simulink library "aerodynamics_lib"  (R2018b)
settings: Solver=VariableStepAuto  StartTime=0.0  StopTime=10.0  RelTol=1e-3
undefined symbols (not defined in the file): copterAero
settings Model: Creator=Ybeyer  LastModifiedBy=yannic
settings SFSimCC: SimUseLocalCustomCode=off
settings RTWCC: RTWUseLocalCustomCode=off
settings CodeAppCC: StateflowObjectComments=on

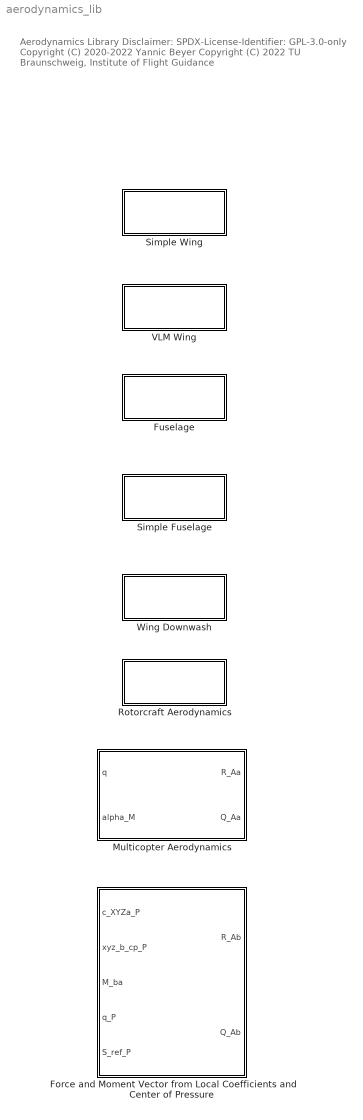
== system aerodynamics_lib ==
  note: Aerodynamics Library
      |
      | Disclaimer:
      | SPDX-License-Identifier: GPL-3.0-only
      |
      | Copyright (C) 2020-2022 Yannic Beyer
      | Copyright (C) 2022 TU Braunschweig, Institute of Flight Guidance
  Force and Moment Vector from Local Coefficients and Center of Pressure : MATLAB Function  TreatAsAtomicUnit=on
  Fuselage : Subsystem
      settings: OpenFcn=fuselage_lib
  Multicopter Aerodynamics : Subsystem  mask{S=copterAero.S, C_D_max=copterAero.C_Dmax, C_D_min=copterAero.C_Dmin, C_L_max=copterAero.C_Lmax, x_CoP_b=copterAero.CoP_xy, z_CoP_b=copterAero.CoP_z}
      mask prompts: S "reference area, m^2"; C_D_max "maximum drag coefficient, -"; C_D_min "minimum drag coefficient, -"; C_L_max "maximum lift coefficient, -"; x_CoP_b "x/y-distance of the center of pressure in body axes, m"; z_CoP_b "z position of the center of pressure in body axes, m"
      mask DialogControl DescGroupVar Prompt: Multicopter Aerodynamics
      mask DialogControl DescTextVar Prompt: This block computes the aerodynamic forces and moments of a simple quadcopter model. Please note that a modified definition of the aerodynamic angles is required.
      mask DialogControl Parameters Prompt: Parameters
  Rotorcraft Aerodynamics : Subsystem
      settings: OpenFcn=rotorcraft_lib
  Simple Fuselage : Subsystem
      settings: OpenFcn=simpleFuselage_lib
  Simple Wing : Subsystem
      settings: OpenFcn=simple_wing_lib
  VLM Wing : Subsystem
      settings: OpenFcn=vlm_wing_lib
  Wing Downwash : Subsystem
      settings: OpenFcn=wing_downwash_lib

== system aerodynamics_lib/Fuselage ==

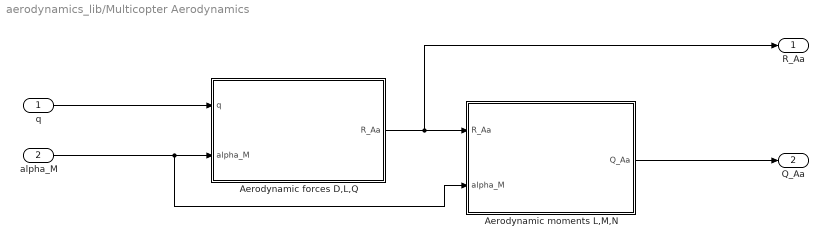
== system aerodynamics_lib/Multicopter Aerodynamics ==
  q : Inport
  alpha_M : Inport  Port=2
  Aerodynamic forces D,L,Q : Subsystem
  Aerodynamic moments L,M,N : Subsystem
  R_Aa : Outport
  Q_Aa : Outport  Port=2
  wires:
  q/1 -> Aerodynamic forces D,L,Q/1(q)
  alpha_M/1 -> Aerodynamic moments L,M,N/2(alpha_M), Aerodynamic forces D,L,Q/2(alpha_M)
  Aerodynamic moments L,M,N/1(Q_Aa) -> Q_Aa/1
  Aerodynamic forces D,L,Q/1(R_Aa) -> R_Aa/1, Aerodynamic moments L,M,N/1(R_Aa)

== system aerodynamics_lib/Rotorcraft Aerodynamics ==

== system aerodynamics_lib/Simple Fuselage ==

== system aerodynamics_lib/Simple Wing ==

== system aerodynamics_lib/VLM Wing ==

== system aerodynamics_lib/Wing Downwash ==

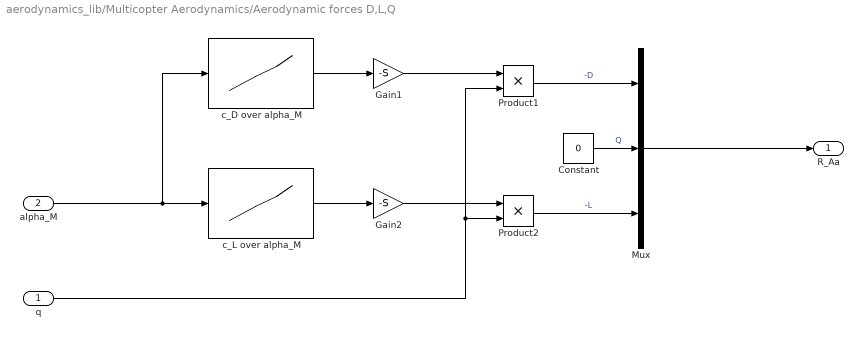
== system aerodynamics_lib/Multicopter Aerodynamics/Aerodynamic forces D,L,Q ==
  q : Inport
  alpha_M : Inport  Port=2
  Constant : Constant  Value=0
  Gain1 : Gain  Gain=-S
  Gain2 : Gain  Gain=-S
  Mux : Mux  Inputs=3
  Product1 : Product
  Product2 : Product
  c_D over alpha_M : Lookup_n-D  NumberOfTableDimensions=1  BreakpointsForDimension1=[-pi/2:pi/50:pi/2]  Table=(C_D_max-C_D_min)/2*-cos(-pi:pi/25:pi)+(C_D_max+C_D_min)/2  InternalRulePriority=Speed  RndMeth=Simplest  InputSameDT=on
  c_L over alpha_M : Lookup_n-D  NumberOfTableDimensions=1  BreakpointsForDimension1=[-pi/2:pi/50:pi/2]  Table=C_L_max*sin(-pi:pi/25:pi)  InternalRulePriority=Speed  RndMeth=Simplest  InputSameDT=on
  R_Aa : Outport
  wires:
  Gain1/1 -> Product1/1
  Mux/1 -> R_Aa/1
  Gain2/1 -> Product2/1
  Product2/1 -> Mux/3  "-L"
  c_D over alpha_M/1 -> Gain1/1
  c_L over alpha_M/1 -> Gain2/1
  alpha_M/1 -> c_D over alpha_M/1, c_L over alpha_M/1
  Product1/1 -> Mux/1  "-D"
  Constant/1 -> Mux/2  "Q"
  q/1 -> Product2/2, Product1/2

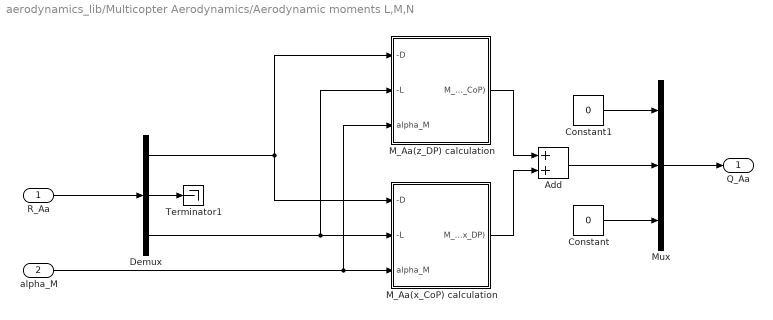
== system aerodynamics_lib/Multicopter Aerodynamics/Aerodynamic moments L,M,N ==
  R_Aa : Inport
  alpha_M : Inport  Port=2
  Add : Sum
  Constant : Constant  Value=0
  Constant1 : Constant  Value=0
  Demux : Demux  Outputs=3
  M_Aa(x_CoP) calculation : Subsystem
  M_Aa(z_DP) calculation : Subsystem
  Mux : Mux  Inputs=3
  Terminator1 : Terminator
  Q_Aa : Outport
  wires:
  Add/1 -> Mux/2
  M_Aa(x_CoP) calculation/1(M_Aa(x_DP)) -> Add/2
  M_Aa(z_DP) calculation/1(M_Aa(z_CoP)) -> Add/1
  Demux/3 -> M_Aa(z_DP) calculation/2(-L), M_Aa(x_CoP) calculation/2(-L)
  alpha_M/1 -> M_Aa(z_DP) calculation/3(alpha_M), M_Aa(x_CoP) calculation/3(alpha_M)
  Demux/1 -> M_Aa(z_DP) calculation/1(-D), M_Aa(x_CoP) calculation/1(-D)
  Demux/2 -> Terminator1/1
  Constant/1 -> Mux/3
  R_Aa/1 -> Demux/1
  Mux/1 -> Q_Aa/1
  Constant1/1 -> Mux/1

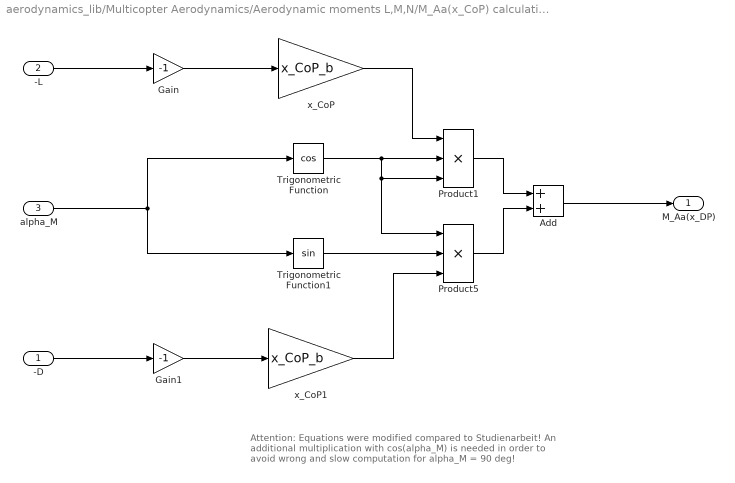
== system aerodynamics_lib/Multicopter Aerodynamics/Aerodynamic moments L,M,N/M_Aa(x_CoP) calculation ==
  note: Attention: Equations were modified compared to Studienarbeit!
      | An additional multiplication with cos(alpha_M) is needed in order
      | to avoid wrong and slow computation for alpha_M = 90 deg!
  -D : Inport
  -L : Inport  Port=2
  alpha_M : Inport  Port=3
  Add : Sum
  Gain : Gain  Gain=-1
  Gain1 : Gain  Gain=-1
  Product1 : Product  Inputs=3
  Product5 : Product  Inputs=3
  Trigonometric Function : Trigonometry  Operator=cos
  Trigonometric Function1 : Trigonometry
  x_CoP : Gain  Gain=x_CoP_b
  x_CoP1 : Gain  Gain=x_CoP_b
  M_Aa(x_DP) : Outport
  wires:
  alpha_M/1 -> Trigonometric Function/1, Trigonometric Function1/1
  -L/1 -> Gain/1
  -D/1 -> Gain1/1
  Product5/1 -> Add/2
  Add/1 -> M_Aa(x_DP)/1
  Product1/1 -> Add/1
  Gain/1 -> x_CoP/1
  Gain1/1 -> x_CoP1/1
  Trigonometric Function/1 -> Product1/2, Product1/3, Product5/1
  Trigonometric Function1/1 -> Product5/2
  x_CoP/1 -> Product1/1
  x_CoP1/1 -> Product5/3

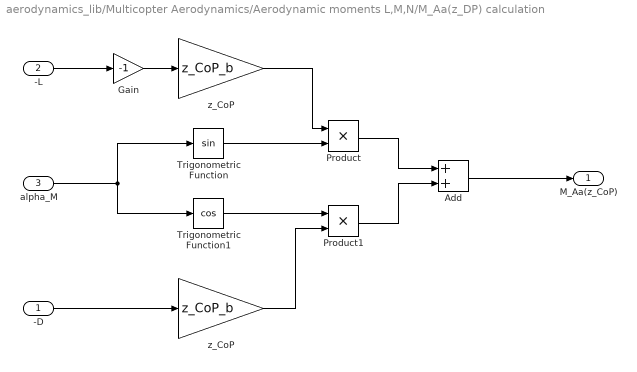
== system aerodynamics_lib/Multicopter Aerodynamics/Aerodynamic moments L,M,N/M_Aa(z_DP) calculation ==
  -D : Inport
  -L : Inport  Port=2
  alpha_M : Inport  Port=3
  Add : Sum
  "Gain " : Gain  Gain=-1
  Product : Product
  Product1 : Product
  Trigonometric Function : Trigonometry
  Trigonometric Function1 : Trigonometry  Operator=cos
  z_CoP : Gain  Gain=z_CoP_b
  "z_CoP " : Gain  Gain=z_CoP_b
  M_Aa(z_CoP) : Outport
  wires:
  -D/1 -> "z_CoP "/1
  -L/1 -> "Gain "/1
  Add/1 -> M_Aa(z_CoP)/1
  "z_CoP "/1 -> Product1/2
  z_CoP/1 -> Product/1
  "Gain "/1 -> z_CoP/1
  Product/1 -> Add/1
  Trigonometric Function/1 -> Product/2
  alpha_M/1 -> Trigonometric Function/1, Trigonometric Function1/1
  Trigonometric Function1/1 -> Product1/1
  Product1/1 -> Add/2

== matlab function aerodynamics_lib/Force and Moment Vector from Local Coefficients and Center of Pressure ==
  data: c_XYZa_P input; R_Ab output; xyz_b_cp_P input; M_ba input; q_P input; S_ref_P input; Q_Ab output
function [ R_Ab, Q_Ab ]  = fcn( c_XYZa_P, xyz_b_cp_P, M_ba, q_P, S_ref_P )
%#codegen

q_P = repmat( q_P, 3, 1 );
S_ref_P = repmat( S_ref_P, 3, 1 );
R_Aa_P = c_XYZa_P.*q_P.*S_ref_P;

R_Ab_P = zeros(3,length(q_P(1,:)));
for i = 1:length(q_P(1,:))
    R_Ab_P(:,i) = M_ba(:,:,i) * R_Aa_P(:,i);
end

% cross product
t1 = [2,3,1]';
t2 = [3,1,2]';
%C = A(:,t1).*B(:,t2)-A(:,t2).*B(:,t1);
Q_Ab_P = xyz_b_cp_P(t1,:).*R_Ab_P(t2,:)-xyz_b_cp_P(t2,:).*R_Ab_P(t1,:);

R_Ab = [sum(R_Ab_P(1,:)); sum(R_Ab_P(2,:)); sum(R_Ab_P(3,:))];
Q_Ab = [sum(Q_Ab_P(1,:)); sum(Q_Ab_P(2,:)); sum(Q_Ab_P(3,:))];
